simulink model "Jb_Model"  (R2023a)
settings: Solver=VariableStepAuto  StartTime=0.0  StopTime=SimulationTime  RelTol=1e-3
values from neighbouring files (symbols this model uses):
  b = J/Taom    [Jb_estimation_DCMotor.m]    (also in parameters.m = 0.000861176470588)
  b_stim = cast(b_stim,"double")    [Jb_estimation_DCMotor.m]
  J = Jm+Jbl    (= 7.32e-05)    [Jb_estimation_DCMotor.m]    (also in parameters.m)
  J_stim = cast(J_stim,"double")    [Jb_estimation_DCMotor.m]
  RadToRpm = 60/(2*pi)    (= 9.54929658551)    [Jb_estimation_DCMotor.m]    (also in parameters.m)
  TSample = 0.0001    [Jb_estimation_DCMotor.m]    (also in parameters.m)
settings Model: Creator=Davide  LastModifiedBy=student
settings DataIOCC: ReturnWorkspaceOutputs=off
settings OptimizationCC: ReuseModelBlockBuffer=off

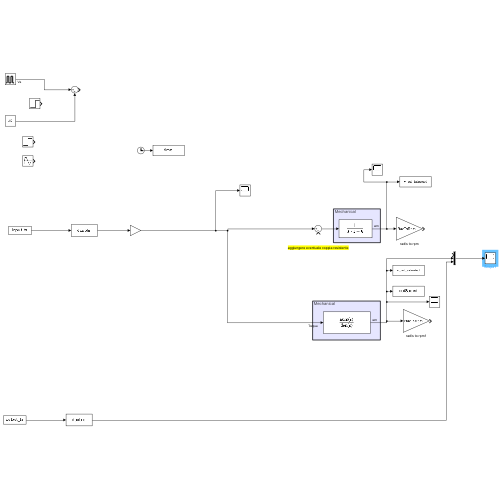
[thumbnail: Simulink's stored preview of the top-level diagram]
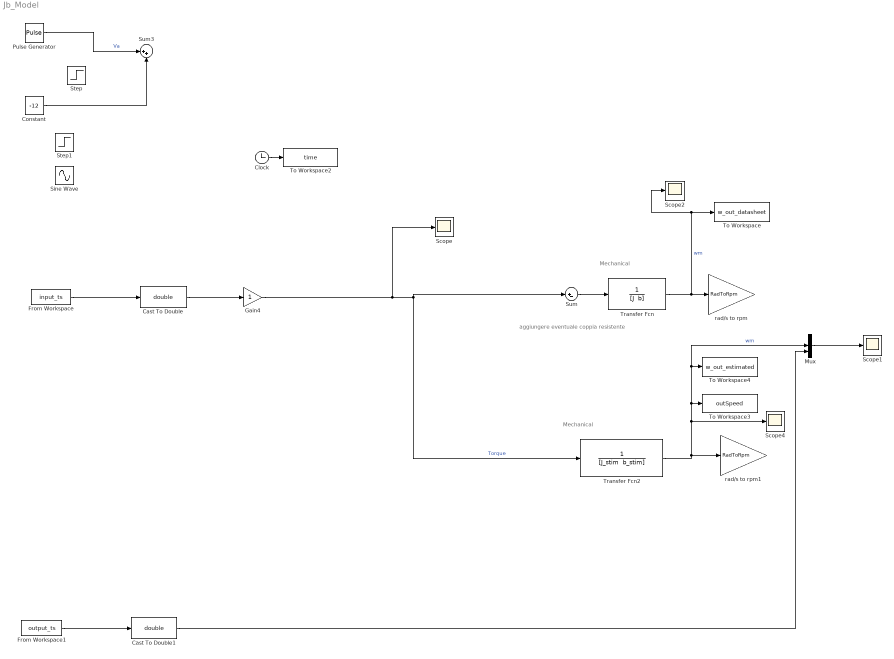
== system Jb_Model ==
  note: aggiungere eventuale coppia resistente
  note: Mechanical
  note: Mechanical
  Cast To Double : DataTypeConversion  OutDataTypeStr=double  SaturateOnIntegerOverflow=off  RndMeth=Floor
  Cast To Double1 : DataTypeConversion  OutDataTypeStr=double  SaturateOnIntegerOverflow=off  RndMeth=Floor
  Clock : Clock
  Constant : Constant  Value=-12
  From Workspace : FromWorkspace  VariableName=input_ts  SampleTime=TSample
  From Workspace1 : FromWorkspace  VariableName=output_ts  SampleTime=TSample
  Gain4 : Gain
  Mux : Mux  Inputs=3
  Pulse Generator : DiscretePulseGenerator  PulseType=Time based  Amplitude=24  Period=1  PulseWidth=20  PhaseDelay=-0.002
  Scope{,1..2,4} (4 alike) : Scope
  Sine Wave : Sin  Amplitude=12  Frequency=150  SampleTime=0
  Step : Step  Time=0  After=24  SampleTime=TSample
  Step1 : Step  Time=0  After=24  SampleTime=TSample
  Sum : Sum  Inputs=|+-
  Sum3 : Sum  Inputs=|++
  To Workspace : ToWorkspace  VariableName=w_out_datasheet  SampleTime=TSample
  To Workspace2 : ToWorkspace  VariableName=time  SampleTime=TSample
  To Workspace3 : ToWorkspace  VariableName=outSpeed  SampleTime=TSample
  To Workspace4 : ToWorkspace  VariableName=w_out_estimated  SampleTime=TSample
  Transfer Fcn : TransferFcn  Denominator="[J  b]"
  Transfer Fcn2 : TransferFcn  Denominator="[J_stim  b_stim]"
  rad/s to rpm : Gain  Gain=RadToRpm  SaturateOnIntegerOverflow=on  OutDataTypeStr=Inherit: Same as input  ParamDataTypeStr=Inherit: Same as input
  rad/s to rpm1 : Gain  Gain=RadToRpm  SaturateOnIntegerOverflow=on  OutDataTypeStr=Inherit: Same as input  ParamDataTypeStr=Inherit: Same as input
  wires:
  Transfer Fcn/1 -> To Workspace/1, Scope2/1, rad/s to rpm/1  "wm"
  Gain4/1 -> Scope/1, Transfer Fcn2/1, Sum/1  "Torque"
  Transfer Fcn2/1 -> Mux/2, To Workspace4/1, To Workspace3/1, Scope4/1, rad/s to rpm1/1  "wm"
  Mux/1 -> Scope1/1
  Sum/1 -> Transfer Fcn/1
  Clock/1 -> To Workspace2/1
  Constant/1 -> Sum3/2
  From Workspace/1 -> Cast To Double/1
  Pulse Generator/1 -> Sum3/1  "Va"
  Cast To Double/1 -> Gain4/1
  From Workspace1/1 -> Cast To Double1/1
  Cast To Double1/1 -> Mux/3
